simulink library "Damper_Nonlinear"  (R2025b)
settings: Solver=VariableStepAuto  StartTime=0.0  StopTime=10.0  RelTol=1e-3
undefined symbols (not defined in the file): Damper
libraries: fl_lib x4, nesl_utility x4, sdl_lib x1
Description:
  | Component of Simscape Vehicle Templates Library
  | 
  | Copyright 2018-2025 The MathWorks, Inc.
settings Model: Creator=smiller  LastModifiedBy=andrei
settings SolverCC: AlgebraicLoopSolver=TrustRegion
settings DataIOCC: ReturnWorkspaceOutputs=off
settings OptimizationCC: ReuseModelBlockBuffer=off
settings DebuggingCC: UnconnectedInputMsg=warning  UnconnectedOutputMsg=warning  UnconnectedLineMsg=warning  ArithmeticOperatorsInVariantConditions=warning
settings ModelReferenceCC: EnableRefExpFcnMdlSchedulingChecks=on
settings SFSimCC: CustomCodeUndefinedFunction=UseInterfaceOnly
settings RTWCC: GPUComputeCapability=3.5  DLArmComputeVersion=19.05

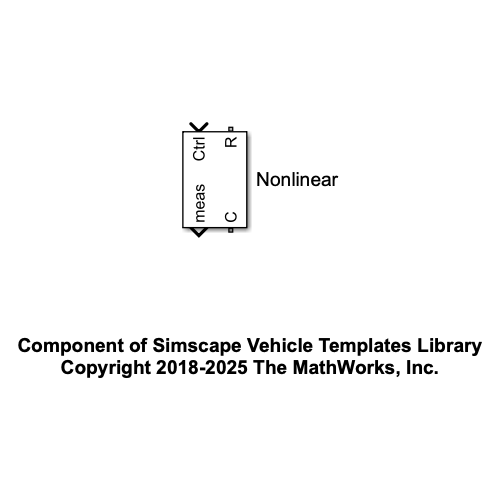
[thumbnail: Simulink's stored preview of the top-level diagram]
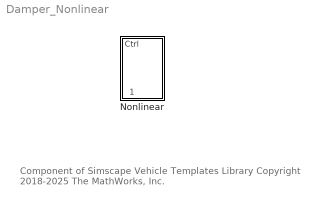
== system Damper_Nonlinear ==
  note: Component of Simscape Vehicle Templates Library
      | Copyright 2018-2025 The MathWorks, Inc.
  Nonlinear : Subsystem  VariantControl=Nonlinear  mask(Nonlinear Damper with Bumpstop){d=Damper.Damping.Value, hp_dpr_top=Damper.Damping.sTop.Value, hp_dpr_bot=Damper.Damping.sBottom.Value, bs_lim_upper=Damper.Endstop.xMax.Value, bs_lim_lower=Damper.Endstop.xMin.Value, bs_k_upper=Damper.KxMax.Value, bs_k_lower=Damper.KxMin.Value, bs_b_upper=Damper.dxMax.Value, bs_b_lower=Damper.dxMin.Value, bs_region=Damper.xTransition.Value}
      mask prompts: d "Damper (N/(m/s))"; hp_dpr_top "HP Damper Top [xyz] (m)"; hp_dpr_bot "HP Damper Bottom [xyz] (m)"; bs_region "Transition Region (m)"
      mask help: Damper with damping coefficient specified as a lookup table in parallel with a bumpstop.
      mask init:
      | dam_x0 = norm(hp_dpr_top - hp_dpr_bot);
      | velocity_vector = d(:, 1)';
      | force_vector = d(:, 2)';
      mask DialogControl text_bumpstop_upper Prompt: Upper
      mask DialogControl text_bumpstop_lower Prompt: Lower
      mask DialogControl text_bumpstop_limit Prompt: Limit (m)
      mask DialogControl text_bumpstop_k Prompt: Stiffness (N/m)
      mask DialogControl text_bumpstop_b Prompt: Damping  (N/(m/s))

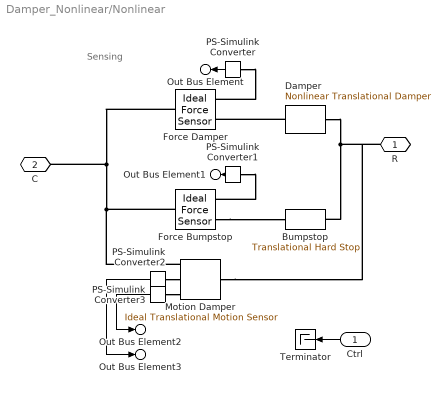
== system Damper_Nonlinear/Nonlinear ==
  note: Sensing
  Ctrl : Inport
  Bumpstop : fl_lib/Mechanical/Translational Elements/Translational Hard Stop  upper_bnd=bs_lim_upper m  lower_bnd=bs_lim_lower m  model=1  stiff_up=bs_k_upper N/m  stiff_low=bs_k_lower N/m  D_up=bs_b_upper N/(m/s)  D_low=bs_b_lower N/(m/s)  transition=bs_region m  coeff_rest=0.7  v_tol=0.001 m/s  f_tol=0.001 N  v_specify=off  v_priority=None  v=0 m/s  v_nominal_specify=off  v_nominal_value=1  v_nominal_unit=m/s  f_specify=off  f_priority=None  f=0 N  f_nominal_specify=off  f_nominal_value=1  f_nominal_unit=N  x_specify=off  x_priority=High  x=0 m  x_nominal_specify=off  x_nominal_value=1  x_nominal_unit=m  M_specify=off  M_priority=None  M=0
  Damper : sdl_lib/Couplings & Drives/Springs & Dampers/Nonlinear Translational Damper  parameterization=sdl.enum.polynomialTLU.tlu  symmetry=1  coefficient_vector=[10, 0, 1, 0, .1] N/(m/s)  extension_coefficient_vector=[10, 0, 1, 0, .1] N/(m/s)  contraction_coefficient_vector=[100, -1, 10, 0, 0] N/(m/s)  velocity_vector=velocity_vector mm/s  force_vector=force_vector N  interp_method=simscape.enum.interpolation.linear  extrap_method=simscape.enum.extrapolation.linear
      settings: InternalSimscapePortConfiguration="{\"Bottom\":[],\"Left\":[{\"id\":\"R\",\"label\":\"R\",\"type\":\"foundation.mechanical.translational.translational\"}],\"Right\":[{\"id\":\"C\",\"label\":\"C\",\"type\":\"foundation.mechanical.translational.translational\"}],\"Top\":[]}"
  Force Bumpstop : fl_lib/Mechanical/Mechanical Sensors/Ideal Force Sensor
  Force Damper : fl_lib/Mechanical/Mechanical Sensors/Ideal Force Sensor
  Motion Damper : fl_lib/Mechanical/Mechanical Sensors/Ideal Translational Motion Sensor  reference=foundation.enum.MeasurementReference.difference  acceleration_port=false  velocity_port=true  position_port=true  offset=dam_x0 m
  PS-Simulink Converter : nesl_utility/PS-Simulink Converter  PhysicalDomain=network_engine_domain  SubClassName=ps_output  LeftPortType=input  RightPortType=output  PseudoPeriodic=off  Frequencies=[]  VectorFormat=1-D array  Unit=N  AffineConversion=off
  PS-Simulink Converter1 : nesl_utility/PS-Simulink Converter  PhysicalDomain=network_engine_domain  SubClassName=ps_output  LeftPortType=input  RightPortType=output  PseudoPeriodic=off  Frequencies=[]  VectorFormat=1-D array  Unit=N  AffineConversion=off
  PS-Simulink Converter2 : nesl_utility/PS-Simulink Converter  PhysicalDomain=network_engine_domain  SubClassName=ps_output  LeftPortType=input  RightPortType=output  PseudoPeriodic=off  Frequencies=[]  VectorFormat=1-D array  Unit=m/s  AffineConversion=off
  PS-Simulink Converter3 : nesl_utility/PS-Simulink Converter  PhysicalDomain=network_engine_domain  SubClassName=ps_output  LeftPortType=input  RightPortType=output  PseudoPeriodic=off  Frequencies=[]  VectorFormat=1-D array  Unit=m  AffineConversion=off
  Terminator : Terminator
  R : PMIOPort  Side=Left
  C : PMIOPort  Port=2  Side=Right
  Out Bus Element : Outport  VectorParamsAs1DForOutWhenUnconnected=off  PortName=meas  Element=FDamper
  Out Bus Element1 : Outport  VectorParamsAs1DForOutWhenUnconnected=off  PortName=meas  Element=FBumpstop
  Out Bus Element2 : Outport  VectorParamsAs1DForOutWhenUnconnected=off  PortName=meas  Element=xDamper
  Out Bus Element3 : Outport  VectorParamsAs1DForOutWhenUnconnected=off  PortName=meas  Element=vDamper
  wires:
  PS-Simulink Converter1/1 -> Out Bus Element1/1
  PS-Simulink Converter3/1 -> Out Bus Element2/1
  PS-Simulink Converter2/1 -> Out Bus Element3/1
  PS-Simulink Converter/1 -> Out Bus Element/1
  Ctrl/1 -> Terminator/1
  connections:
  Damper/LConn1 -- R/RConn1 -- Motion Damper/LConn1 -- Bumpstop/LConn1
  Damper/RConn1 -- Force Damper/RConn1
  Force Bumpstop/RConn1 -- Bumpstop/RConn1
  PS-Simulink Converter/LConn1 -- Force Damper/RConn2
  PS-Simulink Converter3/LConn1 -- Motion Damper/RConn3
  PS-Simulink Converter1/LConn1 -- Force Bumpstop/RConn2
  PS-Simulink Converter2/LConn1 -- Motion Damper/RConn2
  Force Damper/LConn1 -- C/RConn1 -- Force Bumpstop/LConn1 -- Motion Damper/RConn1
